simulink model "turret_digital_twin"  (R2025b)
settings: Solver=ode45  StartTime=0.0  StopTime=10.0  RelTol=1e-4  AbsTol=1e-5
settings Model: Creator=BERKAY  LastModifiedBy=BERKAY

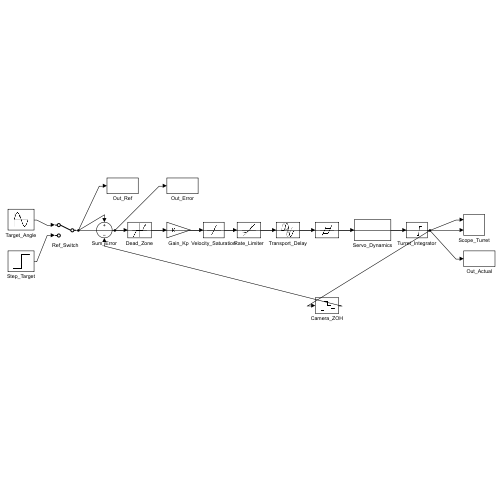
[thumbnail: Simulink's stored preview of the top-level diagram]
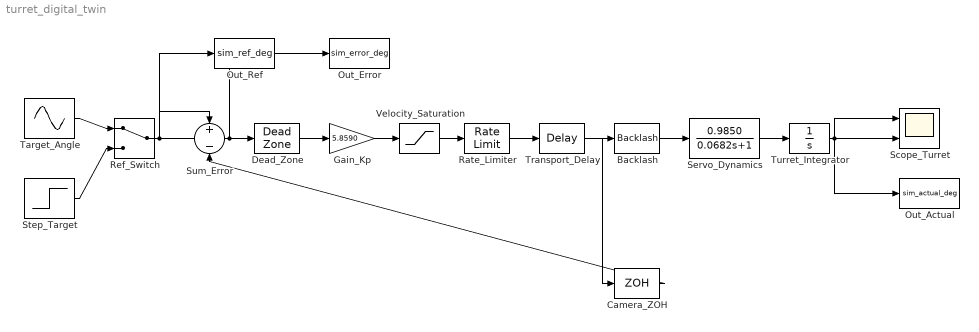
== system turret_digital_twin ==
  Backlash : Backlash  BacklashWidth=1.6100  InitialOutput=0.0
  Camera_ZOH : ZeroOrderHold  SampleTime=0.03333
  Dead_Zone : DeadZone  LowerValue=-0.8500  UpperValue=0.8500
  Gain_Kp : Gain  Gain=5.8590
  Out_Actual : ToWorkspace  VariableName=sim_actual_deg  SaveFormat=Timeseries  SampleTime=-1
  Out_Error : ToWorkspace  VariableName=sim_error_deg  SaveFormat=Timeseries  SampleTime=-1
  Out_Ref : ToWorkspace  VariableName=sim_ref_deg  SaveFormat=Timeseries  SampleTime=-1
  Rate_Limiter : RateLimiter  RisingSlewLimit=353.1  FallingSlewLimit=-353.1  SampleTimeMode=inherited
  Ref_Switch : ManualSwitch
  Scope_Turret : Scope  NumInputPorts=2
  Servo_Dynamics : TransferFcn  Numerator=[0.9850]  Denominator=[0.0682 1]
  Step_Target : Step  Time=1.0  Before=90.0  After=95.0  SampleTime=0
  Sum_Error : Sum  Inputs=+-
  Target_Angle : Sin  Amplitude=10.0  Bias=90.0  Frequency=0.15 * 2 * pi  SampleTime=0
  Transport_Delay : TransportDelay  DelayTime=0.0667  InitialOutput=0.0
  Turret_Integrator : Integrator  InitialCondition=90.0  LimitOutput=on  UpperSaturationLimit=180.0  LowerSaturationLimit=0.0
  Velocity_Saturation : Saturate  UpperLimit=45.0  LowerLimit=-45.0
  wires:
  Target_Angle/1 -> Ref_Switch/1
  Step_Target/1 -> Ref_Switch/2
  Ref_Switch/1 -> Sum_Error/1, Out_Ref/1, Scope_Turret/2
  Sum_Error/1 -> Dead_Zone/1, Out_Error/1
  Dead_Zone/1 -> Gain_Kp/1
  Gain_Kp/1 -> Velocity_Saturation/1
  Velocity_Saturation/1 -> Rate_Limiter/1
  Rate_Limiter/1 -> Transport_Delay/1
  Transport_Delay/1 -> Backlash/1
  Backlash/1 -> Servo_Dynamics/1
  Servo_Dynamics/1 -> Turret_Integrator/1
  Turret_Integrator/1 -> Scope_Turret/1, Out_Actual/1, Camera_ZOH/1
  Camera_ZOH/1 -> Sum_Error/2
